simulink model "MVC27_Sim"  (R2022b)
settings: Solver=FixedStepAuto  StartTime=0.0  StopTime=Sim.Tsim  FixedStep=Sim.Ts  RelTol=1e-3
values from neighbouring files (symbols this model uses):
  g = 9.81    [sim_para.m]
  tdis_FL = 0.3455    [meso_para.m]
  tdis_FR = 0.3455    [meso_para.m]
  tdis_RL = 1 - (tdis_FR + tdis_FL + tdis_RR)    (= 0.1545)    [meso_para.m]
  tdis_RR = 0.1545    [meso_para.m]
undefined symbols (not defined in the file or in its folder): Ctl, DYC, EPS, flag, Motor, Road, Sim, Slip, Steer, Vehicle, Wheel, Wind, WPT
libraries: simulink x3
(part 1 of 2)
settings Model: Creator=takum  LastModifiedBy=nguye
settings DataIOCC: SaveTime=off  ReturnWorkspaceOutputsName=simout
settings OptimizationCC: ReuseModelBlockBuffer=on
settings ModelReferenceCC: EnableRefExpFcnMdlSchedulingChecks=on

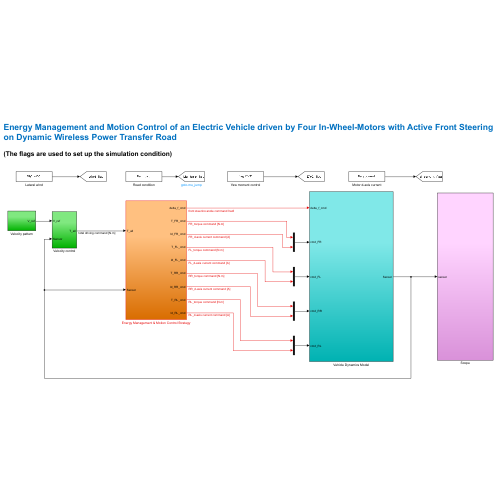
[thumbnail: Simulink's stored preview of the top-level diagram]
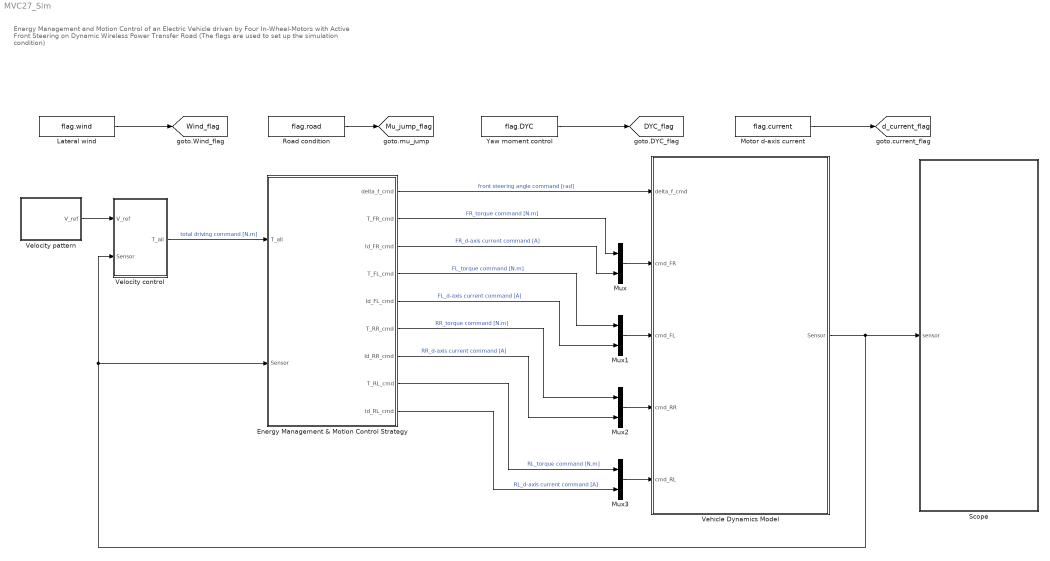
== system MVC27_Sim ==
  note: Energy Management and Motion Control of an Electric Vehicle driven by Four In-Wheel-Motors with Active Front Steering
      | on Dynamic Wireless Power Transfer Road
      |
      | (The flags are used to set up the simulation condition)
  Energy Management & Motion Control Strategy : Subsystem
  Lateral wind : Constant  Value=flag.wind
  Motor d-axis current : Constant  Value=flag.current
  Mux{,1..3} (4 alike) : Mux  Inputs=2
  Road condition : Constant  Value=flag.road
  Scope : Subsystem
  Vehicle Dynamics Model : Subsystem
  Velocity control : Subsystem
  Velocity pattern : Subsystem
  Yaw moment control : Constant  Value=flag.DYC
  tag scope: DYC_flag=global, Mu_jump_flag=global, Wind_flag=global, d_current_flag=global
  wires:
  Mux/1 -> Vehicle Dynamics Model/2(cmd_FR)
  Mux1/1 -> Vehicle Dynamics Model/3(cmd_FL)
  Mux2/1 -> Vehicle Dynamics Model/4(cmd_RR)
  Mux3/1 -> Vehicle Dynamics Model/5(cmd_RL)
  Energy Management & Motion Control Strategy/1(delta_f_cmd) -> Vehicle Dynamics Model/1(delta_f_cmd)  "front steering angle command [rad]"
  Energy Management & Motion Control Strategy/2(T_FR_cmd) -> Mux/1  "FR_torque command [N.m]"
  Energy Management & Motion Control Strategy/3(Id_FR_cmd) -> Mux/2  "FR_d-axis current command [A]"
  Energy Management & Motion Control Strategy/4(T_FL_cmd) -> Mux1/1  "FL_torque command [N.m]"
  Energy Management & Motion Control Strategy/5(Id_FL_cmd) -> Mux1/2  "FL_d-axis current command [A]"
  Energy Management & Motion Control Strategy/6(T_RR_cmd) -> Mux2/1  "RR_torque command [N.m]"
  Energy Management & Motion Control Strategy/7(Id_RR_cmd) -> Mux2/2  "RR_d-axis current command [A]"
  Energy Management & Motion Control Strategy/8(T_RL_cmd) -> Mux3/1  "RL_torque command [N.m]"
  Energy Management & Motion Control Strategy/9(Id_RL_cmd) -> Mux3/2  "RL_d-axis current command [A]"
  Vehicle Dynamics Model/1(Sensor) -> Scope/1(sensor), Energy Management & Motion Control Strategy/2(Sensor), Velocity control/2(Sensor)
  Velocity pattern/1(V_ref) -> Velocity control/1(V_ref)
  Velocity control/1(T_all) -> Energy Management & Motion Control Strategy/1(T_all)  "total driving command [N.m]"
  Yaw moment control/1 -> [DYC_flag]
  Lateral wind/1 -> [Wind_flag]
  Motor d-axis current/1 -> [d_current_flag]
  Road condition/1 -> [Mu_jump_flag]

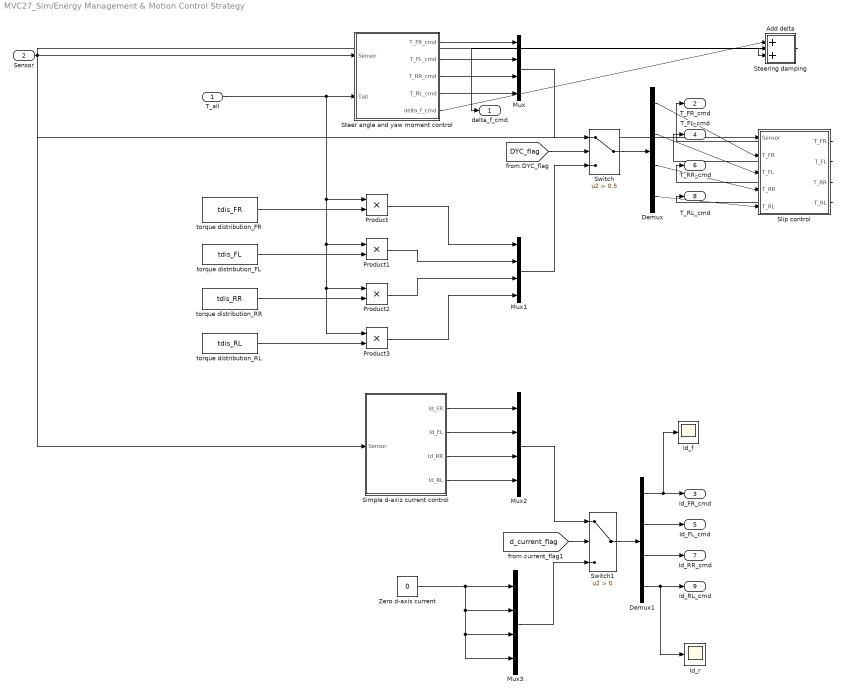
== system MVC27_Sim/Energy Management & Motion Control Strategy ==
  T_all : Inport
  Sensor : Inport  Port=2
  Demux : Demux
  Demux1 : Demux
  Id_f : Scope
  Id_r : Scope
  Mux{,1..3} (4 alike) : Mux
  Product{,1..3} (4 alike) : Product
  Simple d-axis current control : Subsystem
  Steer angle and yaw moment control : Subsystem
  Switch : Switch  Criteria=u2 > Threshold  Threshold=0.5  SaturateOnIntegerOverflow=off  InputSameDT=off
  Switch1 : Switch  Criteria=u2 > Threshold  SaturateOnIntegerOverflow=off  InputSameDT=off
  Zero d-axis current : Constant  Value=0
  torque distribution_FL : Constant  Value=tdis_FL
  torque distribution_FR : Constant  Value=tdis_FR
  torque distribution_RL : Constant  Value=tdis_RL
  torque distribution_RR : Constant  Value=tdis_RR
  delta_f_cmd : Outport
  T_FR_cmd : Outport  Port=2
  Id_FR_cmd : Outport  Port=3
  T_FL_cmd : Outport  Port=4
  Id_FL_cmd : Outport  Port=5
  T_RR_cmd : Outport  Port=6
  Id_RR_cmd : Outport  Port=7
  T_RL_cmd : Outport  Port=8
  Id_RL_cmd : Outport  Port=9
  Slip control : Subsystem
  Steering damping : Subsystem
  Add delta : Sum  Inputs=++
  wires:
  T_all/1 -> Steer angle and yaw moment control/2(Tall), Product/1, Product1/1, Product2/1, Product3/1
  torque distribution_FR/1 -> Product/2
  torque distribution_FL/1 -> Product1/2
  torque distribution_RR/1 -> Product2/2
  torque distribution_RL/1 -> Product3/2
  [DYC_flag] -> Switch/2
  Steer angle and yaw moment control/1(T_FR_cmd) -> Mux/1
  Steer angle and yaw moment control/2(T_FL_cmd) -> Mux/2
  Steer angle and yaw moment control/4(T_RL_cmd) -> Mux/4
  Steer angle and yaw moment control/3(T_RR_cmd) -> Mux/3
  Mux/1 -> Switch/1
  Product/1 -> Mux1/1
  Product3/1 -> Mux1/4
  Product2/1 -> Mux1/3
  Product1/1 -> Mux1/2
  Mux1/1 -> Switch/3
  Switch/1 -> Demux/1
  [d_current_flag] -> Switch1/2
  Simple d-axis current control/1(Id_FR) -> Mux2/1
  Simple d-axis current control/2(Id_FL) -> Mux2/2
  Simple d-axis current control/3(Id_RR) -> Mux2/3
  Simple d-axis current control/4(Id_RL) -> Mux2/4
  Mux2/1 -> Switch1/1
  Mux3/1 -> Switch1/3
  Zero d-axis current/1 -> Mux3/3, Mux3/4, Mux3/2, Mux3/1
  Switch1/1 -> Demux1/1
  Demux1/1 -> Id_f/1, Id_FR_cmd/1
  Demux1/2 -> Id_FL_cmd/1
  Demux1/3 -> Id_RR_cmd/1
  Demux1/4 -> Id_r/1, Id_RL_cmd/1
  Demux/1 -> Slip control/2(T_FR)
  Demux/2 -> Slip control/3(T_FL)
  Demux/3 -> Slip control/4(T_RR)
  Demux/4 -> Slip control/5(T_RL)
  Slip control/1(T_FR) -> T_FR_cmd/1
  Slip control/2(T_FL) -> T_FL_cmd/1
  Slip control/3(T_RR) -> T_RR_cmd/1
  Slip control/4(T_RL) -> T_RL_cmd/1
  Sensor/1 -> Simple d-axis current control/1(Sensor), Steer angle and yaw moment control/1(Sensor), Slip control/1(Sensor), Steering damping/1(Sensor)
  Steer angle and yaw moment control/5(delta_f_cmd) -> Add delta/1
  Steering damping/1(delta_damp) -> Add delta/2
  Add delta/1 -> delta_f_cmd/1

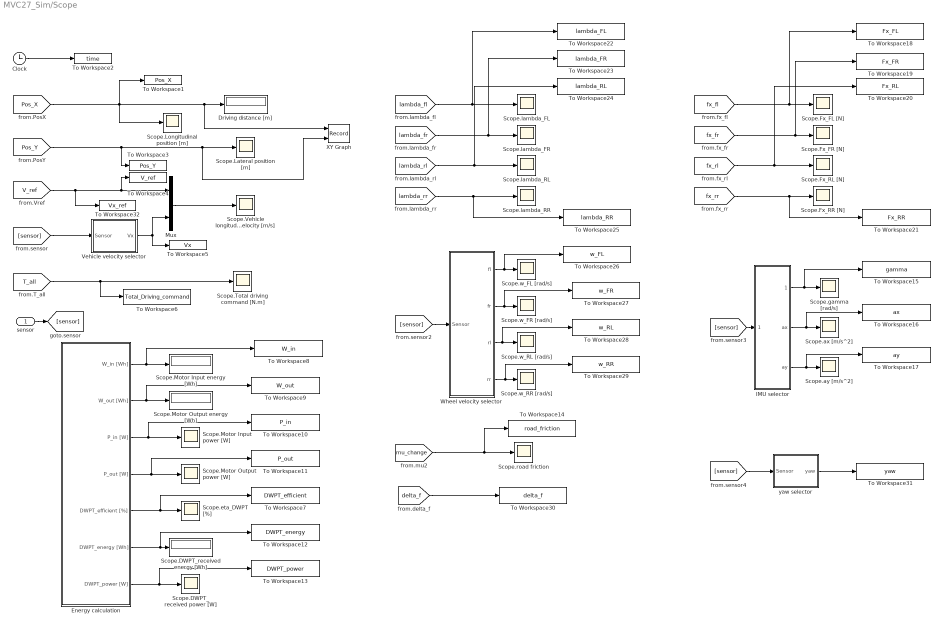
== system MVC27_Sim/Scope ==
  sensor : Inport
  Clock : Clock
  Driving distance [m] : Display
  Energy calculation : Subsystem
  IMU selector : Subsystem
  Mux : Mux  Inputs=2
  Scope.DWPT_received energy [Wh] : Display
  Scope.DWPT_received power [W] : Scope
  Scope.Fx_FL [N] : Scope
  Scope.Fx_FR [N] : Scope
  Scope.Fx_RL [N] : Scope
  Scope.Fx_RR [N] : Scope
  Scope.Lateral position [m] : Scope
  Scope.Longitudinal position [m] : Scope
  Scope.Motor Input energy [Wh] : Display
  Scope.Motor Input power [W] : Scope
  Scope.Motor Output energy [Wh] : Display
  Scope.Motor Output power [W] : Scope
  Scope.Total driving command [N.m] : Scope
  Scope.Vehicle longitudinal velocity [m/s] : Scope
  Scope.ax [m/s^2] : Scope
  Scope.ay [m/s^2] : Scope
  Scope.eta_DWPT [%] : Scope
  Scope.gamma [rad/s] : Scope
  Scope.lambda_FL : Scope
  Scope.lambda_FR : Scope
  Scope.lambda_RL : Scope
  Scope.lambda_RR : Scope
  Scope.road friction : Scope
  Scope.w_FL [rad/s] : Scope
  Scope.w_FR [rad/s] : Scope
  Scope.w_RL [rad/s] : Scope
  Scope.w_RR [rad/s] : Scope
  To Workspace1 : ToWorkspace  VariableName=Pos_X  SampleTime=-1
  To Workspace10 : ToWorkspace  VariableName=P_in  SampleTime=-1
  To Workspace11 : ToWorkspace  VariableName=P_out  SampleTime=-1
  To Workspace12 : ToWorkspace  VariableName=DWPT_energy  SampleTime=-1
  To Workspace13 : ToWorkspace  VariableName=DWPT_power  SampleTime=-1
  To Workspace14 : ToWorkspace  VariableName=road_friction  SampleTime=-1
  To Workspace15 : ToWorkspace  VariableName=gamma  SampleTime=-1
  To Workspace16 : ToWorkspace  VariableName=ax  SampleTime=-1
  To Workspace17 : ToWorkspace  VariableName=ay  SampleTime=-1
  To Workspace18 : ToWorkspace  VariableName=Fx_FL  SampleTime=-1
  To Workspace19 : ToWorkspace  VariableName=Fx_FR  SampleTime=-1
  To Workspace2 : ToWorkspace  VariableName=time  SampleTime=-1
  To Workspace20 : ToWorkspace  VariableName=Fx_RL  SampleTime=-1
  To Workspace21 : ToWorkspace  VariableName=Fx_RR  SampleTime=-1
  To Workspace22 : ToWorkspace  VariableName=lambda_FL  SampleTime=-1
  To Workspace23 : ToWorkspace  VariableName=lambda_FR  SampleTime=-1
  To Workspace24 : ToWorkspace  VariableName=lambda_RL  SampleTime=-1
  To Workspace25 : ToWorkspace  VariableName=lambda_RR  SampleTime=-1
  To Workspace26 : ToWorkspace  VariableName=w_FL  SampleTime=-1
  To Workspace27 : ToWorkspace  VariableName=w_FR  SampleTime=-1
  To Workspace28 : ToWorkspace  VariableName=w_RL  SampleTime=-1
  To Workspace29 : ToWorkspace  VariableName=w_RR  SampleTime=-1
  To Workspace3 : ToWorkspace  VariableName=Pos_Y  SampleTime=-1
  To Workspace30 : ToWorkspace  VariableName=delta_f  SampleTime=-1
  To Workspace31 : ToWorkspace  VariableName=yaw  SampleTime=-1
  To Workspace32 : ToWorkspace  VariableName=Vx_ref  SampleTime=-1
  To Workspace4 : ToWorkspace  VariableName=V_ref  SampleTime=-1
  To Workspace5 : ToWorkspace  VariableName=Vx  SampleTime=-1
  To Workspace6 : ToWorkspace  VariableName=Total_Driving_command  SampleTime=-1
  To Workspace7 : ToWorkspace  VariableName=DWPT_efficient  SampleTime=-1
  To Workspace8 : ToWorkspace  VariableName=W_in  SampleTime=-1
  To Workspace9 : ToWorkspace  VariableName=W_out  SampleTime=-1
  Vehicle velocity selector : Subsystem
  Wheel velocity selector : Subsystem
  XY Graph : Record  FileSettingsInternal="{\"entries\":[{\"content\":{\"excelSettings\":{\"content\":{},\"type\":\"Streamout.ExcelSettings\"}},\"type\":\"Streamout.FileSettingStorage\",\"uuid\":\"\"}],\"packageUris\":[\"http:\\/\\/schema.mathworks.com\\/mf0\\/streamout_blocks\\/R2020a\"],\"version\":\"1.0\"}"  Layout=[1 1]  SignalsInternal="{\"entries\":[{\"content\":{\"signals\":[{\"content\":{\"blockPath\":[],\"channel\":[],\"dimensions\":[1],\"domain\":\"\",\"lineColor\":\"#0072bd\",\"plots\":[],\"port\":1,\"sid\":[],\"signalID\":8,\"signalName\":\"from.PosX\"},\"type\":\"RecordBlkView.Signal\",\"uuid\":\"\"},{\"content\":{\"blockPath\":[],\"channel\":[],\"dimensions\":[1],\"domain\":\"\",\"lineColor\":\"#d95319\",\"plots\":[],\"port\":2,\"sid\":[],\"signalID\":11,\"signalName\":\"from.PosY\"},\"type\":\"RecordBlkView.Signal\",\"uuid\":\"\"}]},\"type\":\"RecordBlkView.InputSignals\",\"uuid\":\"\"}],\"packageUris\":[\"http:\\/\\/schema.mathworks.com\\/mf0\\/streamout_blocks\\/R2020a\"],\"version\":\"1.0\"}"  VisualizationBindings="{\"xyplotplugin\":{\"info\":[{\"series\":[],\"subplotID\":1}]}}"  CompatibilityTag=XY
  yaw selector : Subsystem
  wires:
  [V_ref] -> To Workspace32/1, Mux/1, To Workspace4/1
  Vehicle velocity selector/1(Vx) -> To Workspace5/1, Mux/2
  Mux/1 -> Scope.Vehicle longitudinal velocity [m/s]/1
  Energy calculation/1(W_in [Wh]) -> To Workspace8/1, Scope.Motor Input energy [Wh]/1
  Energy calculation/2(W_out [Wh]) -> To Workspace9/1, Scope.Motor Output energy [Wh]/1
  Energy calculation/3(P_in [W]) -> To Workspace10/1, Scope.Motor Input power [W]/1
  Energy calculation/4(P_out [W]) -> To Workspace11/1, Scope.Motor Output power [W]/1
  [Pos_X] -> To Workspace1/1, Scope.Longitudinal position [m]/1, XY Graph/1, Driving distance [m]/1
  [T_all] -> Scope.Total driving command [N.m]/1, To Workspace6/1
  [lambda_fl] -> To Workspace22/1, Scope.lambda_FL/1
  [lambda_fr] -> To Workspace23/1, Scope.lambda_FR/1
  [lambda_rl] -> To Workspace24/1, Scope.lambda_RL/1
  [lambda_rr] -> To Workspace25/1, Scope.lambda_RR/1
  [fx_fr] -> To Workspace19/1, Scope.Fx_FR [N]/1
  [fx_rr] -> To Workspace21/1, Scope.Fx_RR [N]/1
  [fx_rl] -> Scope.Fx_RL [N]/1, To Workspace20/1
  [fx_fl] -> To Workspace18/1, Scope.Fx_FL [N]/1
  [sensor] -> Wheel velocity selector/1(Sensor)
  sensor/1 -> [sensor]
  [sensor] -> Vehicle velocity selector/1(Sensor)
  Wheel velocity selector/1(fl) -> To Workspace26/1, Scope.w_FL [rad/s]/1
  Wheel velocity selector/2(fr) -> To Workspace27/1, Scope.w_FR [rad/s]/1
  Wheel velocity selector/3(rl) -> To Workspace28/1, Scope.w_RL [rad/s]/1
  Wheel velocity selector/4(rr) -> To Workspace29/1, Scope.w_RR [rad/s]/1
  [sensor] -> IMU selector/1(Sensor)
  [Pos_Y] -> To Workspace3/1, XY Graph/2, Scope.Lateral position [m]/1
  IMU selector/1(gamma) -> To Workspace15/1, Scope.gamma [rad/s]/1
  IMU selector/2(ax) -> To Workspace16/1, Scope.ax [m/s^2]/1
  IMU selector/3(ay) -> To Workspace17/1, Scope.ay [m/s^2]/1
  [mu_change] -> To Workspace14/1, Scope.road friction/1
  Energy calculation/5(DWPT_efficient [%]) -> To Workspace7/1, Scope.eta_DWPT [%]/1
  Energy calculation/6(DWPT_energy [Wh]) -> To Workspace12/1, Scope.DWPT_received energy [Wh]/1
  Energy calculation/7(DWPT_power [W]) -> To Workspace13/1, Scope.DWPT_received power [W]/1
  Clock/1 -> To Workspace2/1
  [delta_f] -> To Workspace30/1
  [sensor] -> yaw selector/1(Sensor)
  yaw selector/1(yaw) -> To Workspace31/1

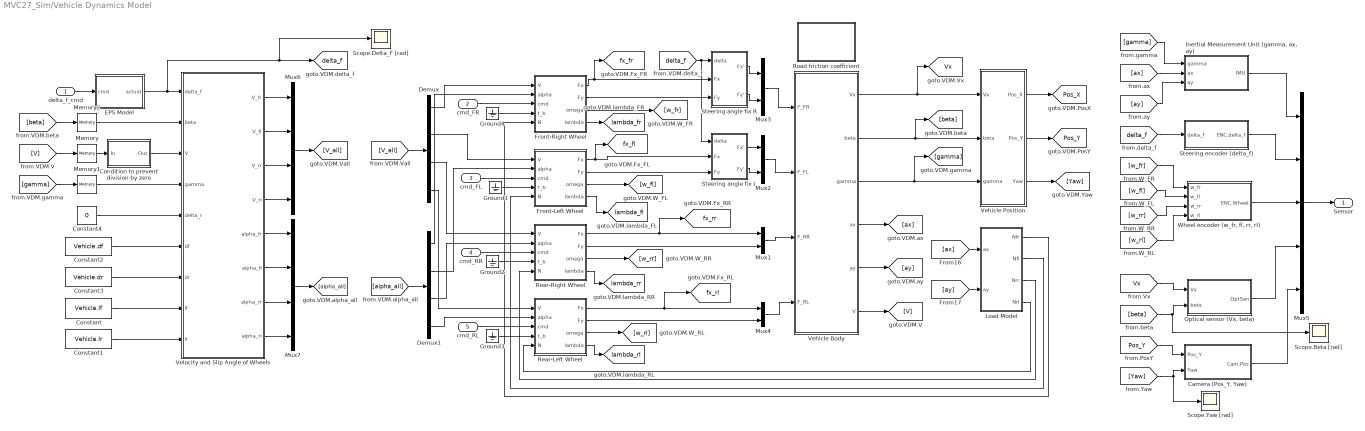
== system MVC27_Sim/Vehicle Dynamics Model ==
  delta_f_cmd : Inport
  cmd_FR : Inport  Port=2
  cmd_FL : Inport  Port=3
  cmd_RR : Inport  Port=4
  cmd_RL : Inport  Port=5
  "Camera (Pos_Y, Yaw)" : Subsystem  TreatAsAtomicUnit=on
  Condition to prevent division by zero : Subsystem  TreatAsAtomicUnit=on
  Constant : Constant  Value=Vehicle.lf
  Constant1 : Constant  Value=Vehicle.lr
  Constant2 : Constant  Value=Vehicle.df
  Constant3 : Constant  Value=Vehicle.dr
  Constant4 : Constant  Value=0
  Demux : Demux
  Demux1 : Demux
  EPS Model : Subsystem
  Front-Left Wheel : Subsystem
  Front-Right Wheel : Subsystem
  Ground{1..4} (4 alike) : Ground
  "Inertial Measurement Unit (gamma, ax, ay)" : Subsystem  TreatAsAtomicUnit=on
  Load Model : Subsystem
  Memory : Memory
  Memory1 : Memory
  Memory2 : Memory
  Mux{1..4} (4 alike) : Mux  Inputs=2
  Mux5 : Mux  Inputs=5
  Mux6 : Mux
  Mux7 : Mux
  "Optical sensor (Vx, beta)" : Subsystem  TreatAsAtomicUnit=on
  Rear-Left Wheel : Subsystem
  Rear-Right Wheel : Subsystem
  Road friction coefficient : Subsystem
  Scope.Beta [rad] : Scope
  Scope.Delta_F [rad] : Scope
  Scope.Yaw [rad] : Scope
  Steering angle fix L : Subsystem
  Steering angle fix R : Subsystem
  Steering encoder (delta_f) : Subsystem  TreatAsAtomicUnit=on
  Vehicle Body : Subsystem
  Vehicle Position : Subsystem
  Velocity and Slip Angle of Wheels : MATLAB Function  TreatAsAtomicUnit=on
  "Wheel encoder (w_fr, fl, rr, rl)" : Subsystem  TreatAsAtomicUnit=on
  Sensor : Outport
  tag scope: Pos_X=global, Pos_Y=global, Vx=global, delta_f=global, fx_fl=global, fx_fr=global, fx_rl=global, fx_rr=global, lambda_fl=global, lambda_fr=global, lambda_rl=global, lambda_rr=global
  wires:
  cmd_FR/1 -> Front-Right Wheel/3(cmd)
  Rear-Right Wheel/1(Fx) -> [fx_rr], Mux1/1
  Rear-Right Wheel/2(Fy) -> Mux1/2
  Rear-Left Wheel/1(Fx) -> [fx_rl], Mux4/1
  Mux3/1 -> Vehicle Body/1(F_FR)
  Mux2/1 -> Vehicle Body/2(F_FL)
  Mux1/1 -> Vehicle Body/3(F_RR)
  Mux4/1 -> Vehicle Body/4(F_RL)
  Vehicle Body/3(gamma) -> [gamma], Vehicle Position/3(gamma)
  Vehicle Body/2(beta) -> [beta], Vehicle Position/2(beta)
  Vehicle Body/1(Vx) -> [Vx], Vehicle Position/1(Vx)
  Vehicle Body/4(ax) -> [ax]
  Vehicle Body/5(ay) -> [ay]
  Load Model/1(Nfr) -> Front-Right Wheel/5(N)
  Load Model/2(Nfl) -> Front-Left Wheel/5(N)
  Load Model/3(Nrr) -> Rear-Right Wheel/5(N)
  Steering angle fix L/1(Fx') -> Mux2/1
  Steering angle fix L/2(Fy') -> Mux2/2
  Steering angle fix R/2(Fy') -> Mux3/2
  Steering angle fix R/1(Fx') -> Mux3/1
  Front-Right Wheel/1(Fx) -> [fx_fr], Steering angle fix R/2(Fx)
  Front-Right Wheel/2(Fy) -> Steering angle fix R/3(Fy)
  Front-Left Wheel/1(Fx) -> [fx_fl], Steering angle fix L/2(Fx)
  Front-Left Wheel/2(Fy) -> Steering angle fix L/3(Fy)
  Ground2/1 -> Rear-Right Wheel/4(t_b)
  Ground3/1 -> Rear-Left Wheel/4(t_b)
  Rear-Left Wheel/2(Fy) -> Mux4/2
  Ground4/1 -> Front-Right Wheel/4(t_b)
  cmd_FL/1 -> Front-Left Wheel/3(cmd)
  Ground1/1 -> Front-Left Wheel/4(t_b)
  cmd_RR/1 -> Rear-Right Wheel/3(cmd)
  cmd_RL/1 -> Rear-Left Wheel/3(cmd)
  Constant2/1 -> Velocity and Slip Angle of Wheels/6(df)
  Constant3/1 -> Velocity and Slip Angle of Wheels/7(dr)
  Constant/1 -> Velocity and Slip Angle of Wheels/8(lf)
  Constant1/1 -> Velocity and Slip Angle of Wheels/9(lr)
  Constant4/1 -> Velocity and Slip Angle of Wheels/5(delta_r)
  Front-Right Wheel/4(lambda) -> [lambda_fr]
  Vehicle Position/1(Pos_X) -> [Pos_X]
  Load Model/4(Nrl) -> Rear-Left Wheel/5(N)
  [gamma] -> "Inertial Measurement Unit (gamma, ax, ay)"/1(gamma)
  [ax] -> "Inertial Measurement Unit (gamma, ax, ay)"/2(ax)
  [ay] -> "Inertial Measurement Unit (gamma, ax, ay)"/3(ay)
  [delta_f] -> Steering encoder (delta_f)/1(delta_f)
  Front-Right Wheel/3(omega) -> [w_fr]
  Front-Left Wheel/3(omega) -> [w_fl]
  Rear-Right Wheel/3(omega) -> [w_rr]
  Rear-Left Wheel/3(omega) -> [w_rl]
  [w_fr] -> "Wheel encoder (w_fr, fl, rr, rl)"/1(w_fr)
  [w_fl] -> "Wheel encoder (w_fr, fl, rr, rl)"/2(w_fl)
  [w_rr] -> "Wheel encoder (w_fr, fl, rr, rl)"/3(w_rr)
  [w_rl] -> "Wheel encoder (w_fr, fl, rr, rl)"/4(w_rl)
  Vehicle Position/2(Pos_Y) -> [Pos_Y]
  Vehicle Position/3(Yaw) -> [Yaw]
  [Vx] -> "Optical sensor (Vx, beta)"/1(Vx)
  [beta] -> Scope.Beta [rad]/1, "Optical sensor (Vx, beta)"/2(beta)
  [Pos_Y] -> "Camera (Pos_Y, Yaw)"/1(Pos_Y)
  [Yaw] -> Scope.Yaw [rad]/1, "Camera (Pos_Y, Yaw)"/2(Yaw)
  "Wheel encoder (w_fr, fl, rr, rl)"/1(ENC.Wheel) -> Mux5/3
  Mux5/1 -> Sensor/1
  "Inertial Measurement Unit (gamma, ax, ay)"/1(IMU) -> Mux5/1
  Steering encoder (delta_f)/1(ENC.delta_f) -> Mux5/2
  "Optical sensor (Vx, beta)"/1(OptSen) -> Mux5/4
  "Camera (Pos_Y, Yaw)"/1(Cam.Pos) -> Mux5/5
  [delta_f] -> Steering angle fix L/1(delta), Steering angle fix R/1(delta)
  Velocity and Slip Angle of Wheels/3(V_rr) -> Mux6/3
  Velocity and Slip Angle of Wheels/2(V_fl) -> Mux6/2
  Velocity and Slip Angle of Wheels/1(V_fr) -> Mux6/1
  Velocity and Slip Angle of Wheels/4(V_rl) -> Mux6/4
  Velocity and Slip Angle of Wheels/8(alpha_rl) -> Mux7/4
  Velocity and Slip Angle of Wheels/7(alpha_rr) -> Mux7/3
  Velocity and Slip Angle of Wheels/6(alpha_fl) -> Mux7/2
  Velocity and Slip Angle of Wheels/5(alpha_fr) -> Mux7/1
  Mux6/1 -> [V_all]
  Mux7/1 -> [alpha_all]
  [V_all] -> Demux/1
  [alpha_all] -> Demux1/1
  Demux/1 -> Front-Right Wheel/1(V)
  Demux/2 -> Front-Left Wheel/1(V)
  Demux/3 -> Rear-Right Wheel/1(V)
  Demux/4 -> Rear-Left Wheel/1(V)
  Demux1/1 -> Front-Right Wheel/2(alpha)
  Demux1/2 -> Front-Left Wheel/2(alpha)
  Demux1/3 -> Rear-Right Wheel/2(alpha)
  Demux1/4 -> Rear-Left Wheel/2(alpha)
  delta_f_cmd/1 -> EPS Model/1(cmd)
  EPS Model/1(actual) -> Scope.Delta_F [rad]/1, [delta_f], Velocity and Slip Angle of Wheels/1(delta_f)
  Memory/1 -> Condition to prevent division by zero/1(In)
  Memory1/1 -> Velocity and Slip Angle of Wheels/4(gamma)
  Memory2/1 -> Velocity and Slip Angle of Wheels/2(beta)
  Vehicle Body/6(V) -> [V]
  [ax] -> Load Model/1(ax)
  [ay] -> Load Model/2(ay)
  [gamma] -> Memory1/1
  [V] -> Memory/1
  [beta] -> Memory2/1
  Condition to prevent division by zero/1(Out) -> Velocity and Slip Angle of Wheels/3(V)
  Rear-Left Wheel/4(lambda) -> [lambda_rl]
  Rear-Right Wheel/4(lambda) -> [lambda_rr]
  Front-Left Wheel/4(lambda) -> [lambda_fl]

== system MVC27_Sim/Velocity control ==
  V_ref : Inport
  Sensor : Inport  Port=2
  Add : Sum  Inputs=+-
  Controller : Subsystem
  Velocity selector : Subsystem
  T_all : Outport
  tag scope: T_all=global, V_ref=global
  wires:
  Sensor/1 -> Velocity selector/1(Sensor)
  V_ref/1 -> [V_ref], Controller/1(V_ref), Add/1
  Velocity selector/1(Vx) -> Add/2
  Controller/1(T_all) -> [T_all], T_all/1
  Add/1 -> Controller/2(Delta_V)

== system MVC27_Sim/Velocity pattern ==
  Add : Sum  Inputs=++-
  Ramp : simulink/Sources/Ramp  slope=2.5  start=0  InitialOutput=0
  Ramp1 : simulink/Sources/Ramp  slope=2.5  start=110  InitialOutput=0
  Ramp2 : simulink/Sources/Ramp  slope=1  start=40  InitialOutput=0
  Saturation : Saturate  UpperLimit=15  LowerLimit=-15
  Saturation1 : Saturate  UpperLimit=20  LowerLimit=-20
  Saturation2 : Saturate  UpperLimit=5  LowerLimit=-5
  V_ref : Outport
  wires:
  Ramp/1 -> Saturation/1
  Saturation/1 -> Add/1
  Ramp1/1 -> Saturation1/1
  Add/1 -> V_ref/1
  Saturation2/1 -> Add/2
  Ramp2/1 -> Saturation2/1
  Saturation1/1 -> Add/3

== system MVC27_Sim/Energy Management & Motion Control Strategy/Simple d-axis current control ==
  Sensor : Inport
  Add1 : Sum
  Add4 : Sum
  Constant1 : Constant  Value=Wheel.R*Wheel.R*Motor.Ra_r*Motor.Rce_r*Motor.Rce_r
  Constant2 : Constant  Value=Wheel.R*Wheel.R*Motor.Ra_f*Motor.Rce_f*Motor.Rce_f
  Divide : Product  Inputs=*/
  Divide1 : Product  Inputs=*/
  Gain : Gain  Gain=Motor.Ld_f*Motor.pn_f
  Gain1 : Gain  Gain=(Motor.Ra_f+Motor.Rce_f)
  Gain2 : Gain  Gain=Motor.pn_f
  Gain3 : Gain  Gain=-(Motor.Ra_f+Motor.Rce_f)*Motor.Ld_f*Motor.Psi_f
  Gain4 : Gain  Gain=Motor.Ld_r*Motor.pn_r
  Gain5 : Gain  Gain=(Motor.Ra_r+Motor.Rce_r)
  Gain6 : Gain  Gain=Motor.pn_r
  Gain7 : Gain  Gain=-(Motor.Ra_r+Motor.Rce_r)*Motor.Ld_r*Motor.Psi_r
  Product{,1..3} (4 alike) : Product
  vehicle speed selector : Subsystem
  Id_FR : Outport
  Id_FL : Outport  Port=2
  Id_RR : Outport  Port=3
  Id_RL : Outport  Port=4
  wires:
  Sensor/1 -> vehicle speed selector/1(Sensor)
  vehicle speed selector/1(Vx) -> [Vx]
  Product1/1 -> Gain3/1
  Gain/1 -> Product/2, Product/1
  Gain3/1 -> Divide/1
  Constant2/1 -> Add4/2
  Gain2/1 -> Product1/2, Product1/1
  Add4/1 -> Divide/2
  Gain1/1 -> Add4/1
  Product/1 -> Gain1/1
  [Vx] -> Gain/1, Gain2/1
  Divide/1 -> Id_FL/1, Id_FR/1
  Add1/1 -> Divide1/2
  Product2/1 -> Gain5/1
  Gain5/1 -> Add1/1
  Gain7/1 -> Divide1/1
  [Vx] -> Gain4/1, Gain6/1
  Product3/1 -> Gain7/1
  Gain6/1 -> Product3/2, Product3/1
  Constant1/1 -> Add1/2
  Gain4/1 -> Product2/2, Product2/1
  Divide1/1 -> Id_RL/1, Id_RR/1

== system MVC27_Sim/Energy Management & Motion Control Strategy/Steer angle and yaw moment control ==
  Sensor : Inport
  Tall : Inport  Port=2
  Add1 : Sum
  Add2 : Sum
  Add3 : Sum  Inputs=+-
  Gain : Gain  Gain=1/4
  Gain1 : Gain  Gain=Wheel.R/(2*Vehicle.d)
  Lateral position and heading angle selector : Subsystem
  Nz : Scope
  steering angle control : Subsystem
  yaw moment control_pos_y : Subsystem  TreatAsAtomicUnit=on
  yaw moment control_yaw : Subsystem  TreatAsAtomicUnit=on
  T_FR_cmd : Outport
  T_FL_cmd : Outport  Port=2
  T_RR_cmd : Outport  Port=3
  T_RL_cmd : Outport  Port=4
  delta_f_cmd : Outport  Port=5
  wires:
  Lateral position and heading angle selector/2(Yaw) -> [yaw]
  [Nz] -> Gain1/1
  Gain1/1 -> Add2/2, Add3/2
  Add2/1 -> T_RR_cmd/1, T_FR_cmd/1
  Add3/1 -> T_RL_cmd/1, T_FL_cmd/1
  Add1/1 -> [Nz], Nz/1
  Gain/1 -> Add3/1, Add2/1
  [PosY] -> steering angle control/1(POS_Y), yaw moment control_pos_y/1(In1)
  [yaw] -> steering angle control/2(Yaw), yaw moment control_yaw/1(In1)
  yaw moment control_pos_y/1(Out1) -> Add1/1
  yaw moment control_yaw/1(Out1) -> Add1/2
  Sensor/1 -> Lateral position and heading angle selector/1(Sensor)
  Tall/1 -> Gain/1
  Lateral position and heading angle selector/1(POS_Y) -> [PosY]
  steering angle control/1(delta_f_cmd) -> delta_f_cmd/1

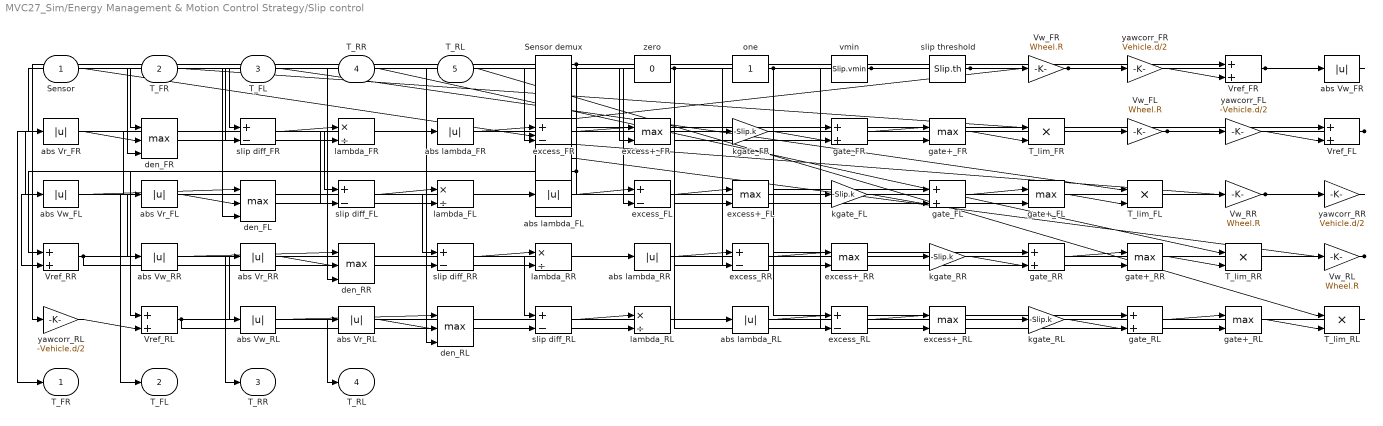
== system MVC27_Sim/Energy Management & Motion Control Strategy/Slip control ==
  Sensor : Inport
  T_FR : Inport  Port=2
  T_FL : Inport  Port=3
  T_RR : Inport  Port=4
  T_RL : Inport  Port=5
  Sensor demux : Demux  Outputs=12
  zero : Constant  Value=0
  one : Constant  Value=1
  vmin : Constant  Value=Slip.vmin
  slip threshold : Constant  Value=Slip.th
  Vw_FR : Gain  Gain=Wheel.R
  yawcorr_FR : Gain  Gain=Vehicle.d/2
  Vref_FR : Sum  Inputs=++
  abs Vw_FR : Abs
  abs Vr_FR : Abs
  den_FR : MinMax  Function=max  Inputs=3
  slip diff_FR : Sum  Inputs=+-
  lambda_FR : Product  Inputs=*/
  abs lambda_FR : Abs
  excess_FR : Sum  Inputs=+-
  excess+_FR : MinMax  Function=max  Inputs=2
  kgate_FR : Gain  Gain=-Slip.k
  gate_FR : Sum  Inputs=++
  gate+_FR : MinMax  Function=max  Inputs=2
  T_lim_FR : Product
  Vw_FL : Gain  Gain=Wheel.R
  yawcorr_FL : Gain  Gain=-Vehicle.d/2
  Vref_FL : Sum  Inputs=++
  abs Vw_FL : Abs
  abs Vr_FL : Abs
  den_FL : MinMax  Function=max  Inputs=3
  slip diff_FL : Sum  Inputs=+-
  lambda_FL : Product  Inputs=*/
  abs lambda_FL : Abs
  excess_FL : Sum  Inputs=+-
  excess+_FL : MinMax  Function=max  Inputs=2
  kgate_FL : Gain  Gain=-Slip.k
  gate_FL : Sum  Inputs=++
  gate+_FL : MinMax  Function=max  Inputs=2
  T_lim_FL : Product
  Vw_RR : Gain  Gain=Wheel.R
  yawcorr_RR : Gain  Gain=Vehicle.d/2
  Vref_RR : Sum  Inputs=++
  abs Vw_RR : Abs
  abs Vr_RR : Abs
  den_RR : MinMax  Function=max  Inputs=3
  slip diff_RR : Sum  Inputs=+-
  lambda_RR : Product  Inputs=*/
  abs lambda_RR : Abs
  excess_RR : Sum  Inputs=+-
  excess+_RR : MinMax  Function=max  Inputs=2
  kgate_RR : Gain  Gain=-Slip.k
  gate_RR : Sum  Inputs=++
  gate+_RR : MinMax  Function=max  Inputs=2
  T_lim_RR : Product
  Vw_RL : Gain  Gain=Wheel.R
  yawcorr_RL : Gain  Gain=-Vehicle.d/2
  Vref_RL : Sum  Inputs=++
  abs Vw_RL : Abs
  abs Vr_RL : Abs
  den_RL : MinMax  Function=max  Inputs=3
  slip diff_RL : Sum  Inputs=+-
  lambda_RL : Product  Inputs=*/
  abs lambda_RL : Abs
  excess_RL : Sum  Inputs=+-
  excess+_RL : MinMax  Function=max  Inputs=2
  kgate_RL : Gain  Gain=-Slip.k
  gate_RL : Sum  Inputs=++
  gate+_RL : MinMax  Function=max  Inputs=2
  T_lim_RL : Product
  T_FR : Outport
  T_FL : Outport  Port=2
  T_RR : Outport  Port=3
  T_RL : Outport  Port=4
  wires:
  Sensor/1 -> Sensor demux/1
  Sensor demux/5 -> Vw_FR/1
  Sensor demux/1 -> yawcorr_FR/1, yawcorr_FL/1, yawcorr_RR/1, yawcorr_RL/1
  Sensor demux/9 -> Vref_FR/1, Vref_FL/1, Vref_RR/1, Vref_RL/1
  yawcorr_FR/1 -> Vref_FR/2
  Vw_FR/1 -> abs Vw_FR/1, slip diff_FR/1
  Vref_FR/1 -> abs Vr_FR/1, slip diff_FR/2
  abs Vw_FR/1 -> den_FR/1
  abs Vr_FR/1 -> den_FR/2
  vmin/1 -> den_FR/3, den_FL/3, den_RR/3, den_RL/3
  slip diff_FR/1 -> lambda_FR/1
  den_FR/1 -> lambda_FR/2
  lambda_FR/1 -> abs lambda_FR/1
  abs lambda_FR/1 -> excess_FR/1
  slip threshold/1 -> excess_FR/2, excess_FL/2, excess_RR/2, excess_RL/2
  excess_FR/1 -> excess+_FR/1
  zero/1 -> excess+_FR/2, gate+_FR/2, excess+_FL/2, gate+_FL/2, excess+_RR/2, gate+_RR/2, excess+_RL/2, gate+_RL/2
  excess+_FR/1 -> kgate_FR/1
  one/1 -> gate_FR/1, gate_FL/1, gate_RR/1, gate_RL/1
  kgate_FR/1 -> gate_FR/2
  gate_FR/1 -> gate+_FR/1
  T_FR/1 -> T_lim_FR/1
  gate+_FR/1 -> T_lim_FR/2
  Sensor demux/6 -> Vw_FL/1
  yawcorr_FL/1 -> Vref_FL/2
  Vw_FL/1 -> abs Vw_FL/1, slip diff_FL/1
  Vref_FL/1 -> abs Vr_FL/1, slip diff_FL/2
  abs Vw_FL/1 -> den_FL/1
  abs Vr_FL/1 -> den_FL/2
  slip diff_FL/1 -> lambda_FL/1
  den_FL/1 -> lambda_FL/2
  lambda_FL/1 -> abs lambda_FL/1
  abs lambda_FL/1 -> excess_FL/1
  excess_FL/1 -> excess+_FL/1
  excess+_FL/1 -> kgate_FL/1
  kgate_FL/1 -> gate_FL/2
  gate_FL/1 -> gate+_FL/1
  T_FL/1 -> T_lim_FL/1
  gate+_FL/1 -> T_lim_FL/2
  Sensor demux/7 -> Vw_RR/1
  yawcorr_RR/1 -> Vref_RR/2
  Vw_RR/1 -> abs Vw_RR/1, slip diff_RR/1
  Vref_RR/1 -> abs Vr_RR/1, slip diff_RR/2
  abs Vw_RR/1 -> den_RR/1
  abs Vr_RR/1 -> den_RR/2
  slip diff_RR/1 -> lambda_RR/1
  den_RR/1 -> lambda_RR/2
  lambda_RR/1 -> abs lambda_RR/1
  abs lambda_RR/1 -> excess_RR/1
  excess_RR/1 -> excess+_RR/1
  excess+_RR/1 -> kgate_RR/1
  kgate_RR/1 -> gate_RR/2
  gate_RR/1 -> gate+_RR/1
  T_RR/1 -> T_lim_RR/1
  gate+_RR/1 -> T_lim_RR/2
  Sensor demux/8 -> Vw_RL/1
  yawcorr_RL/1 -> Vref_RL/2
  Vw_RL/1 -> abs Vw_RL/1, slip diff_RL/1
  Vref_RL/1 -> abs Vr_RL/1, slip diff_RL/2
  abs Vw_RL/1 -> den_RL/1
  abs Vr_RL/1 -> den_RL/2
  slip diff_RL/1 -> lambda_RL/1
  den_RL/1 -> lambda_RL/2
  lambda_RL/1 -> abs lambda_RL/1
  abs lambda_RL/1 -> excess_RL/1
  excess_RL/1 -> excess+_RL/1
  excess+_RL/1 -> kgate_RL/1
  kgate_RL/1 -> gate_RL/2
  gate_RL/1 -> gate+_RL/1
  T_RL/1 -> T_lim_RL/1
  gate+_RL/1 -> T_lim_RL/2
  T_lim_FR/1 -> T_FR/1
  T_lim_FL/1 -> T_FL/1
  T_lim_RR/1 -> T_RR/1
  T_lim_RL/1 -> T_RL/1

== system MVC27_Sim/Energy Management & Motion Control Strategy/Steering damping ==
  Sensor : Inport
  Sensor demux : Demux  Outputs=12
  yaw rate damping : Gain  Gain=-Steer.Kd
  delta_damp : Outport
  wires:
  Sensor/1 -> Sensor demux/1
  Sensor demux/1 -> yaw rate damping/1
  yaw rate damping/1 -> delta_damp/1

== system MVC27_Sim/Scope/Energy calculation ==
  % cal : Gain  Gain=100
  Add : Sum  Inputs=++++
  Add1 : Sum  Inputs=++++
  DWPT efficiency map : MATLAB Function  TreatAsAtomicUnit=on
  Gain1 : Gain  Gain=1/(3600)
  Gain2 : Gain  Gain=1/(3600)
  Gain6 : Gain  Gain=1/(3600)
  Integrator : Integrator
  Integrator1 : Integrator
  Integrator2 : Integrator
  Longitudinal misalignment : MATLAB Function  TreatAsAtomicUnit=on
  Scope : Scope  NumInputPorts=4
  delta_x [mm] : Scope
  delta_y [mm] : Scope
  m to mm : Gain  Gain=1000
  "m to mm " : Gain  Gain=1000
  power cal : Gain  Gain=WPT.P
  W_in [Wh] : Outport
  W_out [Wh] : Outport  Port=2
  P_in [W] : Outport  Port=3
  P_out [W] : Outport  Port=4
  DWPT_efficient [%] : Outport  Port=5
  DWPT_energy [Wh] : Outport  Port=6
  DWPT_power [W] : Outport  Port=7
  wires:
  [Pin_FR] -> Scope/1, Add/1
  [Pin_FL] -> Scope/2, Add/2
  [Pin_RR] -> Scope/3, Add/3
  [Pin_RL] -> Add/4, Scope/4
  [Pout_FR] -> Add1/1
  [Pout_FL] -> Add1/2
  [Pout_RR] -> Add1/3
  [Pout_RL] -> Add1/4
  Add/1 -> Integrator/1, P_in [W]/1
  Add1/1 -> Integrator1/1, P_out [W]/1
  Integrator/1 -> Gain6/1
  Gain6/1 -> W_in [Wh]/1
  Integrator1/1 -> Gain1/1
  Gain1/1 -> W_out [Wh]/1
  m to mm/1 -> DWPT efficiency map/1(u1), delta_x [mm]/1
  [Pos_Y] -> "m to mm "/1
  [Pos_X] -> Longitudinal misalignment/1(u)
  Longitudinal misalignment/1(y) -> m to mm/1
  "m to mm "/1 -> DWPT efficiency map/2(u2), delta_y [mm]/1
  DWPT efficiency map/1(y) -> power cal/1, % cal/1
  % cal/1 -> DWPT_efficient [%]/1
  power cal/1 -> DWPT_power [W]/1, Integrator2/1
  Integrator2/1 -> Gain2/1
  Gain2/1 -> DWPT_energy [Wh]/1

== system MVC27_Sim/Scope/IMU selector ==
  Sensor : Inport
  Demux : Demux  Outputs=12
  Terminator{2..10} (9 alike) : Terminator
  gamma : Outport
  ax : Outport  Port=2
  ay : Outport  Port=3
  wires:
  Sensor/1 -> Demux/1
  Demux/1 -> gamma/1
  Demux/2 -> ax/1
  Demux/4 -> Terminator3/1
  Demux/5 -> Terminator4/1
  Demux/6 -> Terminator5/1
  Demux/7 -> Terminator6/1
  Demux/8 -> Terminator7/1
  Demux/10 -> Terminator8/1
  Demux/11 -> Terminator9/1
  Demux/12 -> Terminator10/1
  Demux/9 -> Terminator2/1
  Demux/3 -> ay/1

== system MVC27_Sim/Scope/Vehicle velocity selector ==
  Sensor : Inport
  Demux : Demux  Outputs=12
  Terminator{,1..10} (11 alike) : Terminator
  Vx : Outport
  wires:
  Sensor/1 -> Demux/1
  Demux/9 -> Vx/1
  Demux/1 -> Terminator/1
  Demux/2 -> Terminator1/1
  Demux/3 -> Terminator2/1
  Demux/4 -> Terminator3/1
  Demux/5 -> Terminator4/1
  Demux/6 -> Terminator5/1
  Demux/7 -> Terminator6/1
  Demux/8 -> Terminator7/1
  Demux/10 -> Terminator8/1
  Demux/11 -> Terminator9/1
  Demux/12 -> Terminator10/1

== system MVC27_Sim/Scope/Wheel velocity selector ==
  Sensor : Inport
  Demux : Demux  Outputs=12
  Terminator{,1..3,7..10} (8 alike) : Terminator
  fl : Outport
  fr : Outport  Port=2
  rl : Outport  Port=3
  rr : Outport  Port=4
  wires:
  Sensor/1 -> Demux/1
  Demux/1 -> Terminator/1
  Demux/2 -> Terminator1/1
  Demux/3 -> Terminator2/1
  Demux/4 -> Terminator3/1
  Demux/10 -> Terminator8/1
  Demux/11 -> Terminator9/1
  Demux/12 -> Terminator10/1
  Demux/9 -> Terminator7/1
  Demux/5 -> fr/1
  Demux/6 -> fl/1
  Demux/7 -> rr/1
  Demux/8 -> rl/1

== system MVC27_Sim/Scope/yaw selector ==
  Sensor : Inport
  Demux : Demux  Outputs=12
  Terminator{,1..10} (11 alike) : Terminator
  yaw : Outport
  wires:
  Sensor/1 -> Demux/1
  Demux/1 -> Terminator/1
  Demux/2 -> Terminator1/1
  Demux/3 -> Terminator2/1
  Demux/4 -> Terminator3/1
  Demux/5 -> Terminator4/1
  Demux/6 -> Terminator5/1
  Demux/7 -> Terminator6/1
  Demux/8 -> Terminator7/1
  Demux/10 -> Terminator9/1
  Demux/11 -> Terminator10/1
  Demux/12 -> yaw/1
  Demux/9 -> Terminator8/1

== system MVC27_Sim/Vehicle Dynamics Model/Camera (Pos_Y, Yaw) ==
  Pos_Y : Inport
  Yaw : Inport  Port=2
  Mux7 : Mux  Inputs=2
  Cam.Pos : Outport
  wires:
  Pos_Y/1 -> Mux7/1
  Yaw/1 -> Mux7/2
  Mux7/1 -> Cam.Pos/1

== system MVC27_Sim/Vehicle Dynamics Model/Condition to prevent division by zero ==
  In : Inport
  Constant : Constant  Value=0.1
  Switch : Switch  Criteria=u2 > Threshold  Threshold=0.1  SaturateOnIntegerOverflow=off  InputSameDT=off
  Out : Outport
  wires:
  In/1 -> Switch/1, Switch/2
  Constant/1 -> Switch/3
  Switch/1 -> Out/1

== system MVC27_Sim/Vehicle Dynamics Model/EPS Model ==
  cmd : Inport
  Saturation : Saturate  UpperLimit=EPS.Del_max  LowerLimit=-EPS.Del_max
  Transfer Fcn : TransferFcn  Denominator=[EPS.tau 1]
  actual : Outport
  wires:
  cmd/1 -> Transfer Fcn/1
  Transfer Fcn/1 -> Saturation/1
  Saturation/1 -> actual/1

== system MVC27_Sim/Vehicle Dynamics Model/Front-Left Wheel ==
  V : Inport
  alpha : Inport  Port=2
  cmd : Inport  Port=3
  t_b : Inport  Port=4
  N : Inport  Port=5
  Gain4 : Gain  Gain=Wheel.R  SaturateOnIntegerOverflow=on  OutDataTypeStr=Inherit: Same as input  ParamDataTypeStr=Inherit: Same as input
  Memory : Memory
  Motor : Subsystem
  Tire force model : Subsystem  TreatAsAtomicUnit=on
  Fx : Outport
  Fy : Outport  Port=2
  omega : Outport  Port=3
  lambda : Outport  Port=4
  tag scope: Pin_FL=global, Pout_FL=global
  wires:
  Gain4/1 -> Tire force model/2(Vw)
  [mu_FL] -> Tire force model/4(mu)
  N/1 -> Tire force model/5(Fz)
  alpha/1 -> Tire force model/3(alpha)
  V/1 -> Tire force model/1(V)
  cmd/1 -> Motor/1(cmd)
  Tire force model/3(lambda) -> lambda/1
  t_b/1 -> Motor/2(tb)
  Motor/1(omega) -> omega/1, Gain4/1
  Motor/2(Pin) -> [Pin_FL]
  Motor/3(Pout) -> [Pout_FL]
  Tire force model/1(Fx) -> Memory/1, Fx/1
  Tire force model/2(Fy) -> Fy/1
  Memory/1 -> Motor/3(Fx)

== system MVC27_Sim/Vehicle Dynamics Model/Front-Right Wheel ==
  V : Inport
  alpha : Inport  Port=2
  cmd : Inport  Port=3
  t_b : Inport  Port=4
  N : Inport  Port=5
  Gain4 : Gain  Gain=Wheel.R  SaturateOnIntegerOverflow=on  OutDataTypeStr=Inherit: Same as input  ParamDataTypeStr=Inherit: Same as input
  Memory : Memory
  Motor : Subsystem
  Tire force model : Subsystem  TreatAsAtomicUnit=on
  Fx : Outport
  Fy : Outport  Port=2
  omega : Outport  Port=3
  lambda : Outport  Port=4
  tag scope: Pin_FR=global, Pout_FR=global
  wires:
  Gain4/1 -> Tire force model/2(Vw)
  [mu_FR] -> Tire force model/4(mu)
  N/1 -> Tire force model/5(Fz)
  alpha/1 -> Tire force model/3(alpha)
  V/1 -> Tire force model/1(V)
  cmd/1 -> Motor/1(cmd)
  Tire force model/3(lambda) -> lambda/1
  t_b/1 -> Motor/2(tb)
  Motor/1(omega) -> omega/1, Gain4/1
  Motor/2(Pin) -> [Pin_FR]
  Motor/3(Pout) -> [Pout_FR]
  Tire force model/2(Fy) -> Fy/1
  Memory/1 -> Motor/3(Fx)
  Tire force model/1(Fx) -> Memory/1, Fx/1

== system MVC27_Sim/Vehicle Dynamics Model/Inertial Measurement Unit (gamma, ax, ay) ==
  gamma : Inport
  ax : Inport  Port=2
  ay : Inport  Port=3
  Mux7 : Mux  Inputs=3
  IMU : Outport
  wires:
  gamma/1 -> Mux7/1
  ax/1 -> Mux7/2
  ay/1 -> Mux7/3
  Mux7/1 -> IMU/1

== system MVC27_Sim/Vehicle Dynamics Model/Load Model ==
  ax : Inport
  ay : Inport  Port=2
  Gain1 : Gain  Gain=Vehicle.M*Vehicle.hg/(2*Vehicle.l)  SaturateOnIntegerOverflow=on  OutDataTypeStr=Inherit: Same as input  ParamDataTypeStr=Inherit: Same as input
  Gain2 : Gain  Gain=Vehicle.M*(Vehicle.hg/Vehicle.d)*(Vehicle.lf/Vehicle.l)  SaturateOnIntegerOverflow=on  OutDataTypeStr=Inherit: Same as input  ParamDataTypeStr=Inherit: Same as input
  Gain7 : Gain  Gain=Vehicle.M*(Vehicle.hg/Vehicle.d)*(Vehicle.lr/Vehicle.l)  SaturateOnIntegerOverflow=on  OutDataTypeStr=Inherit: Same as input  ParamDataTypeStr=Inherit: Same as input
  Memory1 : Memory  InheritSampleTime=on  LinearizeMemory=on
  Memory2 : Memory
  Static Load_Front : Constant  Value=Vehicle.Nf
  Static Load_Rear : Constant  Value=Vehicle.Nr
  Sum12 : Sum  Inputs=+-+  SaturateOnIntegerOverflow=on
  Sum4 : Sum  Inputs=++-  SaturateOnIntegerOverflow=on
  Sum5 : Sum  Inputs=+--  SaturateOnIntegerOverflow=on
  Sum7 : Sum  Inputs=+++  SaturateOnIntegerOverflow=on
  Nfr : Outport
  Nfl : Outport  Port=2
  Nrr : Outport  Port=3
  Nrl : Outport  Port=4
  wires:
  Gain2/1 -> Sum7/2, Sum12/2
  Gain7/1 -> Sum5/2, Sum4/2
  Static Load_Front/1 -> Sum5/1, Sum4/1
  Sum4/1 -> Nfr/1
  Sum5/1 -> Nfl/1
  Sum12/1 -> Nrl/1
  Sum7/1 -> Nrr/1
  Static Load_Rear/1 -> Sum12/3, Sum7/3
  ay/1 -> Memory1/1
  ax/1 -> Memory2/1
  Memory1/1 -> Gain2/1, Gain7/1
  Gain1/1 -> Sum4/3, Sum12/1, Sum7/1, Sum5/3
  Memory2/1 -> Gain1/1

== system MVC27_Sim/Vehicle Dynamics Model/Optical sensor (Vx, beta) ==
  Vx : Inport
  beta : Inport  Port=2
  Mux7 : Mux  Inputs=2
  OptSen : Outport
  wires:
  Vx/1 -> Mux7/1
  beta/1 -> Mux7/2
  Mux7/1 -> OptSen/1

== system MVC27_Sim/Vehicle Dynamics Model/Rear-Left Wheel ==
  V : Inport
  alpha : Inport  Port=2
  cmd : Inport  Port=3
  t_b : Inport  Port=4
  N : Inport  Port=5
  Gain4 : Gain  Gain=Wheel.R  SaturateOnIntegerOverflow=on  OutDataTypeStr=Inherit: Same as input  ParamDataTypeStr=Inherit: Same as input
  Memory : Memory
  Motor : Subsystem
  Tire force model : Subsystem  TreatAsAtomicUnit=on
  scope.fz : Scope
  Fx : Outport
  Fy : Outport  Port=2
  omega : Outport  Port=3
  lambda : Outport  Port=4
  tag scope: Pin_RL=global, Pout_RL=global
  wires:
  Gain4/1 -> Tire force model/2(Vw)
  alpha/1 -> Tire force model/3(alpha)
  V/1 -> Tire force model/1(V)
  cmd/1 -> Motor/1(cmd)
  Tire force model/3(lambda) -> lambda/1
  t_b/1 -> Motor/2(tb)
  Motor/1(omega) -> omega/1, Gain4/1
  Motor/2(Pin) -> [Pin_RL]
  Motor/3(Pout) -> [Pout_RL]
  Memory/1 -> Motor/3(Fx)
  N/1 -> scope.fz/1, Tire force model/5(Fz)
  Tire force model/2(Fy) -> Fy/1
  Tire force model/1(Fx) -> Memory/1, Fx/1
  [mu_RL] -> Tire force model/4(mu)

== system MVC27_Sim/Vehicle Dynamics Model/Rear-Right Wheel ==
  V : Inport
  alpha : Inport  Port=2
  cmd : Inport  Port=3
  t_b : Inport  Port=4
  N : Inport  Port=5
  Gain4 : Gain  Gain=Wheel.R  SaturateOnIntegerOverflow=on  OutDataTypeStr=Inherit: Same as input  ParamDataTypeStr=Inherit: Same as input
  Memory : Memory
  Motor : Subsystem
  Tire force model : Subsystem  TreatAsAtomicUnit=on
  Fx : Outport
  Fy : Outport  Port=2
  omega : Outport  Port=3
  lambda : Outport  Port=4
  tag scope: Pin_RR=global, Pout_RR=global
  wires:
  Gain4/1 -> Tire force model/2(Vw)
  [mu_RR] -> Tire force model/4(mu)
  N/1 -> Tire force model/5(Fz)
  alpha/1 -> Tire force model/3(alpha)
  V/1 -> Tire force model/1(V)
  cmd/1 -> Motor/1(cmd)
  Tire force model/3(lambda) -> lambda/1
  t_b/1 -> Motor/2(tb)
  Motor/1(omega) -> omega/1, Gain4/1
  Motor/2(Pin) -> [Pin_RR]
  Motor/3(Pout) -> [Pout_RR]
  Tire force model/1(Fx) -> Memory/1, Fx/1
  Tire force model/2(Fy) -> Fy/1
  Memory/1 -> Motor/3(Fx)

== system MVC27_Sim/Vehicle Dynamics Model/Road friction coefficient ==
  Constant : Constant  Value=Road.Mu_l
  Constant{1..2,7,9} (4 alike) : Constant  Value=Road.Mu_h
  Constant8 : Constant  Value=Road.Mu_m
  Switch : Switch  Criteria=u2 > Threshold  Threshold=Road.L_in  SaturateOnIntegerOverflow=off  InputSameDT=off
  Switch1 : Switch  Criteria=u2 > Threshold  Threshold=Road.L_out  SaturateOnIntegerOverflow=off  InputSameDT=off
  Switch2 : Switch  Criteria=u2 > Threshold  Threshold=Road.M_in  SaturateOnIntegerOverflow=off  InputSameDT=off
  Switch3 : Switch  Criteria=u2 > Threshold  Threshold=Road.M_out  SaturateOnIntegerOverflow=off  InputSameDT=off
  Switch4 : Switch  Criteria=u2 > Threshold  Threshold=0.5  SaturateOnIntegerOverflow=off  InputSameDT=off
  tag scope: mu_FL=global, mu_FR=global, mu_RL=global, mu_RR=global, mu_change=global
  wires:
  Constant1/1 -> Switch/3
  Constant/1 -> Switch/1
  Switch/1 -> Switch1/3
  [Pos_X] -> Switch1/2
  Switch2/1 -> Switch3/3
  Constant7/1 -> Switch1/1
  Switch1/1 -> Switch2/3
  Constant8/1 -> Switch2/1
  Constant9/1 -> Switch3/1
  Switch3/1 -> Switch4/1
  [Mu_jump_flag] -> Switch4/2
  Constant2/1 -> Switch4/3
  Switch4/1 -> [mu_RL], [mu_RR], [mu_FR], [mu_FL], [mu_change]
  [Pos_X] -> Switch/2
  [Pos_X] -> Switch2/2
  [Pos_X] -> Switch3/2

== system MVC27_Sim/Vehicle Dynamics Model/Steering angle fix L ==
  delta : Inport
  Fx : Inport  Port=2
  Fy : Inport  Port=3
  Product{1..4} (4 alike) : Product  SaturateOnIntegerOverflow=on  OutDataTypeStr=Inherit: Same as first input
  Sum : Sum  Inputs=+-|  SaturateOnIntegerOverflow=on
  Sum1 : Sum  Inputs=|++  SaturateOnIntegerOverflow=on
  Trigonometric Function1 : Trigonometry  Operator=cos
  Trigonometric Function2 : Trigonometry
  Fx' : Outport
  Fy' : Outport  Port=2
  wires:
  Sum1/1 -> Fy'/1
  delta/1 -> Trigonometric Function2/1, Trigonometric Function1/1
  Fx/1 -> Product1/2, Product3/2
  Trigonometric Function1/1 -> Product4/1, Product1/1
  Fy/1 -> Product4/2, Product2/2
  Trigonometric Function2/1 -> Product2/1, Product3/1
  Product1/1 -> Sum/1
  Product2/1 -> Sum/2
  Sum/1 -> Fx'/1
  Product3/1 -> Sum1/1
  Product4/1 -> Sum1/2

== system MVC27_Sim/Vehicle Dynamics Model/Steering angle fix R ==
  delta : Inport
  Fx : Inport  Port=2
  Fy : Inport  Port=3
  Product{1..4} (4 alike) : Product  SaturateOnIntegerOverflow=on  OutDataTypeStr=Inherit: Same as first input
  Sum : Sum  Inputs=+-|  SaturateOnIntegerOverflow=on
  Sum1 : Sum  Inputs=|++  SaturateOnIntegerOverflow=on
  Trigonometric Function1 : Trigonometry  Operator=cos
  Trigonometric Function2 : Trigonometry
  Fx' : Outport
  Fy' : Outport  Port=2
  wires:
  Product4/1 -> Sum1/2
  Product3/1 -> Sum1/1
  Sum/1 -> Fx'/1
  Product2/1 -> Sum/2
  Product1/1 -> Sum/1
  Trigonometric Function2/1 -> Product3/1, Product2/1
  Fy/1 -> Product2/2, Product4/2
  Trigonometric Function1/1 -> Product1/1, Product4/1
  Fx/1 -> Product3/2, Product1/2
  delta/1 -> Trigonometric Function1/1, Trigonometric Function2/1
  Sum1/1 -> Fy'/1

== system MVC27_Sim/Vehicle Dynamics Model/Steering encoder (delta_f) ==
  delta_f : Inport
  ENC.delta_f : Outport
  wires:
  delta_f/1 -> ENC.delta_f/1

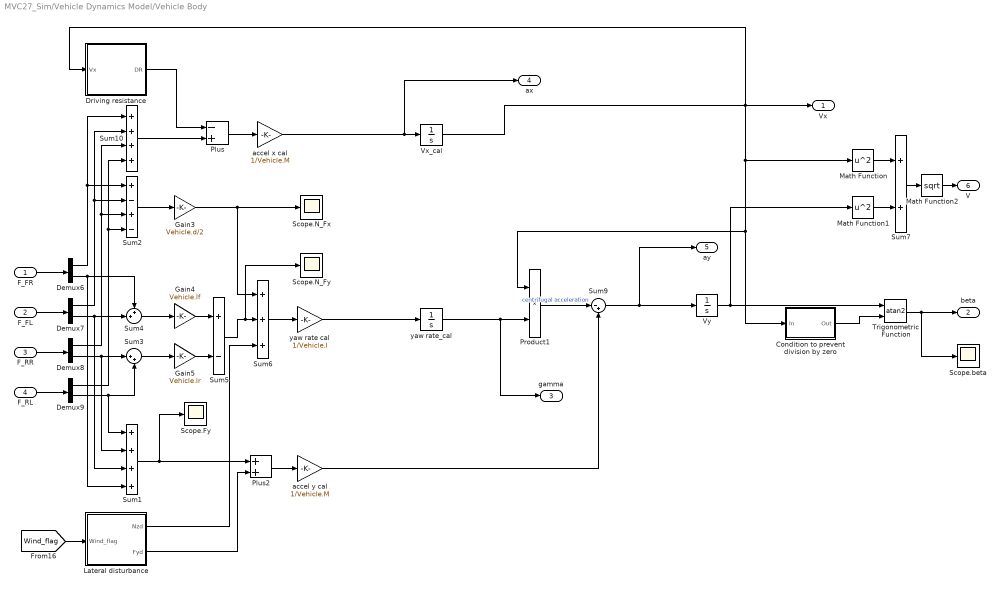
== system MVC27_Sim/Vehicle Dynamics Model/Vehicle Body ==
  F_FR : Inport
  F_FL : Inport  Port=2
  F_RR : Inport  Port=3
  F_RL : Inport  Port=4
  Condition to prevent division by zero : Subsystem  TreatAsAtomicUnit=on
  Demux{6..9} (4 alike) : Demux  Outputs=2
      settings: DisplayOption=none
  Driving resistance : Subsystem  TreatAsAtomicUnit=on
  Gain3 : Gain  Gain=Vehicle.d/2  SaturateOnIntegerOverflow=on  OutDataTypeStr=Inherit: Same as input  ParamDataTypeStr=Inherit: Same as input
  Gain4 : Gain  Gain=Vehicle.lf  SaturateOnIntegerOverflow=on  OutDataTypeStr=Inherit: Same as input  ParamDataTypeStr=Inherit: Same as input
  Gain5 : Gain  Gain=Vehicle.lr  SaturateOnIntegerOverflow=on  OutDataTypeStr=Inherit: Same as input  ParamDataTypeStr=Inherit: Same as input
  Lateral disturbance : Subsystem  TreatAsAtomicUnit=on
  Math Function : Math  Operator=square  SignedPower=on
  Math Function1 : Math  Operator=square  SignedPower=on
  Math Function2 : Math  Operator=sqrt  SignedPower=on
  Plus : Sum  Inputs=-+
  Plus2 : Sum
  Product1 : Product  SaturateOnIntegerOverflow=on  OutDataTypeStr=Inherit: Same as first input
  Scope.Fy : Scope
  Scope.N_Fx : Scope
  Scope.N_Fy : Scope
  Scope.beta : Scope
  Sum1 : Sum  Inputs=4  SaturateOnIntegerOverflow=on
  Sum10 : Sum  Inputs=4  SaturateOnIntegerOverflow=on
  Sum2 : Sum  Inputs=+-+-  SaturateOnIntegerOverflow=on
  Sum3 : Sum  Inputs=|++  SaturateOnIntegerOverflow=on
  Sum4 : Sum  Inputs=++|  SaturateOnIntegerOverflow=on
  Sum5 : Sum  Inputs=+-  SaturateOnIntegerOverflow=on
  Sum6 : Sum  Inputs=+++  SaturateOnIntegerOverflow=on
  Sum7 : Sum  SaturateOnIntegerOverflow=on
  Sum9 : Sum  Inputs=|-+  SaturateOnIntegerOverflow=on
  Trigonometric Function : Trigonometry  Operator=atan2
  Vx_cal : Integrator  InitialCondition=Sim.Ini_V
  Vy : Integrator
  accel x cal : Gain  Gain=1/Vehicle.M  SaturateOnIntegerOverflow=on  OutDataTypeStr=Inherit: Same as input  ParamDataTypeStr=Inherit: Same as input
  accel y cal : Gain  Gain=1/Vehicle.M  SaturateOnIntegerOverflow=on  OutDataTypeStr=Inherit: Same as input  ParamDataTypeStr=Inherit: Same as input
  yaw rate cal : Gain  Gain=1/Vehicle.I  SaturateOnIntegerOverflow=on  OutDataTypeStr=Inherit: Same as input  ParamDataTypeStr=Inherit: Same as input
  yaw rate_cal : Integrator  InitialCondition=Sim.Ini_YR
  Vx : Outport
  beta : Outport  Port=2
  gamma : Outport  Port=3
  ax : Outport  Port=4
  ay : Outport  Port=5
  V : Outport  Port=6
  wires:
  Trigonometric Function/1 -> Scope.beta/1, beta/1
  Vy/1 -> Math Function1/1, Trigonometric Function/1
  Gain3/1 -> Scope.N_Fx/1, Sum6/1
  Product1/1 -> Sum9/1  "centrifugal acceleration"
  Plus/1 -> accel x cal/1
  Sum6/1 -> yaw rate cal/1
  Sum2/1 -> Gain3/1
  Gain4/1 -> Sum5/1
  Demux9/1 -> Sum2/4, Sum10/4
  Demux8/1 -> Sum2/3, Sum10/3
  Demux7/1 -> Sum2/2, Sum10/2
  Demux6/1 -> Sum2/1, Sum10/1
  Gain5/1 -> Sum5/2
  Sum3/1 -> Gain5/1
  Sum4/1 -> Gain4/1
  Demux6/2 -> Sum1/4, Sum4/1
  Demux7/2 -> Sum1/3, Sum4/2
  Demux8/2 -> Sum1/2, Sum3/1
  Demux9/2 -> Sum1/1, Sum3/2
  Sum5/1 -> Scope.N_Fy/1, Sum6/2
  Sum10/1 -> Plus/2
  Sum1/1 -> Scope.Fy/1, Plus2/1
  Plus2/1 -> accel y cal/1
  F_FR/1 -> Demux6/1
  F_FL/1 -> Demux7/1
  F_RR/1 -> Demux8/1
  F_RL/1 -> Demux9/1
  yaw rate_cal/1 -> gamma/1, Product1/2
  Sum9/1 -> Vy/1, ay/1
  Lateral disturbance/1(Nzd) -> Sum6/3
  Lateral disturbance/2(Fyd) -> Plus2/2
  Math Function1/1 -> Sum7/2
  Math Function/1 -> Sum7/1
  Sum7/1 -> Math Function2/1
  Math Function2/1 -> V/1
  Vx_cal/1 -> Math Function/1, Condition to prevent division by zero/1(In), Product1/1, Driving resistance/1(Vx), Vx/1
  Condition to prevent division by zero/1(Out) -> Trigonometric Function/2
  Driving resistance/1(DR) -> Plus/1
  accel x cal/1 -> ax/1, Vx_cal/1
  yaw rate cal/1 -> yaw rate_cal/1
  accel y cal/1 -> Sum9/2
  [Wind_flag] -> Lateral disturbance/1(Wind_flag)

== system MVC27_Sim/Vehicle Dynamics Model/Vehicle Position ==
  Vx : Inport
  beta : Inport  Port=2
  gamma : Inport  Port=3
  Ini_X : Constant  Value=Sim.Ini_X
  Ini_Y : Constant  Value=Sim.Ini_Y
  Ini_Yaw : Constant  Value=Sim.Ini_Yaw
  Integrator : Integrator
  Integrator1 : Integrator
  Integrator2 : Integrator
  Product3 : Product  SaturateOnIntegerOverflow=on  OutDataTypeStr=Inherit: Same as first input
  Product4 : Product  SaturateOnIntegerOverflow=on  OutDataTypeStr=Inherit: Same as first input
  Sum : Sum  Inputs=++|  SaturateOnIntegerOverflow=on
  Sum1 : Sum  Inputs=++|  SaturateOnIntegerOverflow=on
  Sum2 : Sum  Inputs=|++  SaturateOnIntegerOverflow=on
  Sum3 : Sum  Inputs=|++  SaturateOnIntegerOverflow=on
  Trigonometric Function : Trigonometry  Operator=cos
  Trigonometric Function1 : Trigonometry
  Pos_X : Outport
  Pos_Y : Outport  Port=2
  Yaw : Outport  Port=3
  wires:
  gamma/1 -> Integrator/1
  Vx/1 -> Product4/1, Product3/1
  beta/1 -> Sum/1
  Ini_X/1 -> Sum1/1
  Product4/1 -> Integrator1/1
  Sum2/1 -> Pos_Y/1
  Ini_Y/1 -> Sum2/2
  Trigonometric Function1/1 -> Product3/2
  Product3/1 -> Integrator2/1
  Sum1/1 -> Pos_X/1
  Trigonometric Function/1 -> Product4/2
  Sum/1 -> Trigonometric Function/1, Trigonometric Function1/1
  Ini_Yaw/1 -> Sum3/2
  Integrator/1 -> Sum3/1
  Sum3/1 -> Yaw/1, Sum/2
  Integrator1/1 -> Sum1/2
  Integrator2/1 -> Sum2/1

== system MVC27_Sim/Vehicle Dynamics Model/Wheel encoder (w_fr, fl, rr, rl) ==
  w_fr : Inport
  w_fl : Inport  Port=2
  w_rr : Inport  Port=3
  w_rl : Inport  Port=4
  Mux7 : Mux
  ENC.Wheel : Outport
  wires:
  w_fr/1 -> Mux7/1
  w_fl/1 -> Mux7/2
  w_rr/1 -> Mux7/3
  w_rl/1 -> Mux7/4
  Mux7/1 -> ENC.Wheel/1

== system MVC27_Sim/Velocity control/Controller ==
  V_ref : Inport
  Delta_V : Inport  Port=2
  Add : Sum
  Add1 : Sum
  Feed forward control : TransferFcn  Numerator=[Vehicle.M 0]  Denominator=[Ctl.tau_ff_v 1]
  Feedback control gain Ki : Gain  Gain=Ctl.Ki_v
  Feedback control gain Kp : Gain  Gain=Ctl.Kp_v
  Force limitation : Saturate  UpperLimit=Ctl.Fmax  LowerLimit=-Ctl.Fmax
  Gain : Gain  Gain=Wheel.R
  Integrator : Integrator
  T_all : Outport
  wires:
  Delta_V/1 -> Feedback control gain Ki/1, Feedback control gain Kp/1
  Feedback control gain Ki/1 -> Integrator/1
  Feedback control gain Kp/1 -> Add/1
  Integrator/1 -> Add/2
  Add/1 -> Add1/2
  V_ref/1 -> Feed forward control/1
  Add1/1 -> Force limitation/1
  Gain/1 -> T_all/1
  Force limitation/1 -> Gain/1
  Feed forward control/1 -> Add1/1

== system MVC27_Sim/Velocity control/Velocity selector ==
  Sensor : Inport
  Demux : Demux  Outputs=12
  Terminator{,1..10} (11 alike) : Terminator
  Vx : Outport
  wires:
  Sensor/1 -> Demux/1
  Demux/9 -> Vx/1
  Demux/1 -> Terminator/1
  Demux/2 -> Terminator1/1
  Demux/3 -> Terminator2/1
  Demux/4 -> Terminator3/1
  Demux/5 -> Terminator4/1
  Demux/6 -> Terminator5/1
  Demux/7 -> Terminator6/1
  Demux/8 -> Terminator7/1
  Demux/10 -> Terminator8/1
  Demux/11 -> Terminator9/1
  Demux/12 -> Terminator10/1

== system MVC27_Sim/Energy Management & Motion Control Strategy/Simple d-axis current control/vehicle speed selector ==
  Sensor : Inport
  Demux : Demux  Outputs=12
  Terminator{,1..10} (11 alike) : Terminator
  Vx : Outport
  wires:
  Sensor/1 -> Demux/1
  Demux/1 -> Terminator/1
  Demux/2 -> Terminator1/1
  Demux/3 -> Terminator2/1
  Demux/4 -> Terminator3/1
  Demux/10 -> Terminator9/1
  Demux/11 -> Terminator7/1
  Demux/12 -> Terminator6/1
  Demux/8 -> Terminator8/1
  Demux/5 -> Terminator4/1
  Demux/6 -> Terminator5/1
  Demux/7 -> Terminator10/1
  Demux/9 -> Vx/1

== system MVC27_Sim/Energy Management & Motion Control Strategy/Steer angle and yaw moment control/Lateral position and heading angle selector ==
  Sensor : Inport
  Demux : Demux  Outputs=12
  Terminator{,1..9} (10 alike) : Terminator
  POS_Y : Outport
  Yaw : Outport  Port=2
  wires:
  Sensor/1 -> Demux/1
  Demux/1 -> Terminator/1
  Demux/2 -> Terminator1/1
  Demux/3 -> Terminator2/1
  Demux/4 -> Terminator3/1
  Demux/5 -> Terminator4/1
  Demux/6 -> Terminator5/1
  Demux/7 -> Terminator6/1
  Demux/8 -> Terminator7/1
  Demux/12 -> Yaw/1
  Demux/10 -> Terminator9/1
  Demux/9 -> Terminator8/1
  Demux/11 -> POS_Y/1
